simulink model "buck_no_ideal"  (R2024b)
settings: Solver=VariableStepAuto  StartTime=0.0  StopTime=0.59999999999999987  MaxStep=5.0000000000000004e-06  RelTol=1e-3
values from neighbouring files (symbols this model uses):
  C = p(2)    [p6_identificar_ft.m]
  Rs = buck.Rs    [p6_identificar_ft.m]
undefined symbols (not defined in the file or in its folder): fsw, L_inv, L_sat, m_inv, vd, vin, vsw
libraries: simulink x1
settings Model: Creator=pablo  LastModifiedBy=tomas
settings OptimizationCC: ReuseModelBlockBuffer=off
settings RTWCC: GPUComputeCapability=3.5

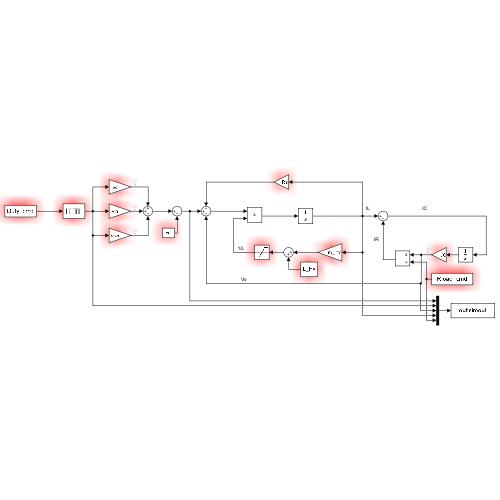
[thumbnail: Simulink's stored preview of the top-level diagram]
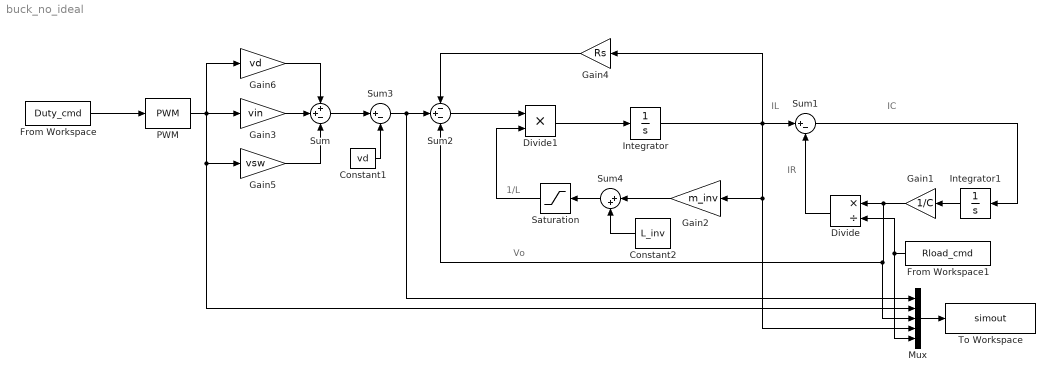
== system buck_no_ideal ==
  note: IL
  note: IC
  note: IR
  note: Vo
  note: 1/L
  Constant1 : Constant  Value=vd
  Constant2 : Constant  Value=L_inv
  Divide : Product  Inputs=*/
  Divide1 : Product  Inputs=**
  From Workspace : FromWorkspace  VariableName=Duty_cmd
  From Workspace1 : FromWorkspace  VariableName=Rload_cmd
  Gain1 : Gain  Gain=1/C
  Gain2 : Gain  Gain=m_inv
  Gain3 : Gain  Gain=vin
  Gain4 : Gain  Gain=Rs
  Gain5 : Gain  Gain=vsw
  Gain6 : Gain  Gain=vd
  Integrator : Integrator  InitialCondition=1.2642667518025357  LowerSaturationLimit=0
  Integrator1 : Integrator  InitialCondition=0.056000949455098287
  Mux : Mux  Inputs=5
  PWM : simulink/Discontinuities/PWM  DisableCoverage=on  Period=1/fsw  InitialDelay=0  DisallowZeroDutyCycle=off  RunAtFixedTimeIntervals=off  SampleTime=0.1
  Saturation : Saturate  UpperLimit=inf  LowerLimit=1/L_sat
  Sum : Sum  Inputs=++-
  Sum1 : Sum  Inputs=|+-
  Sum2 : Sum  Inputs=-+-
  Sum3 : Sum  Inputs=|+-
  Sum4 : Sum  Inputs=|++
  To Workspace : ToWorkspace  VariableName=simout  SampleTime=-1
      settings: Save2DSignal=2-D array (concatenate along first dimension)
  wires:
  Sum1/1 -> Integrator1/1
  Integrator1/1 -> Gain1/1
  Gain1/1 -> Divide/1, Mux/3, Sum2/3
  Divide/1 -> Sum1/2
  PWM/1 -> Gain6/1, Mux/2, Gain5/1, Gain3/1
  From Workspace/1 -> PWM/1
  Mux/1 -> To Workspace/1
  Gain3/1 -> Sum/2
  Gain4/1 -> Sum2/1
  Gain5/1 -> Sum/3
  Sum/1 -> Sum3/1
  Sum3/1 -> Mux/1, Sum2/2
  Gain6/1 -> Sum/1
  Constant1/1 -> Sum3/2
  From Workspace1/1 -> Mux/5, Divide/2
  Sum2/1 -> Divide1/1
  Gain2/1 -> Sum4/1
  Constant2/1 -> Sum4/2
  Integrator/1 -> Gain4/1, Sum1/1, Gain2/1, Mux/4
  Divide1/1 -> Integrator/1
  Sum4/1 -> Saturation/1
  Saturation/1 -> Divide1/2
